simulink library "Multibody_Parts_Lib"  (R2024a)
settings: Solver=VariableStepAuto  StartTime=0.0  StopTime=10.0  RelTol=1e-3
undefined symbols (not defined in the file or in its folder): b_gear_pd_asy, b_radius_asy, b_visc_frict_asy, bevel_angle_asy, bevel_angle_bf_asy, bevel_angle_fg_asy, f_gear_pd_asy, f_radius_asy, f_visc_frict_asy, g_radius_asy, g_visc_frict_asy, gear_ra_asy, gear_visc_frict_asy, Hand, Left, Local, pinion_pd_asy, screw_lead, worm_lead_angle_asy, worm_rad_asy, worm_visc_frict_asy, X, Y, Z
libraries: sm_lib x143, $bdroot x22, nesl_utility x16
(part 4 of 6)

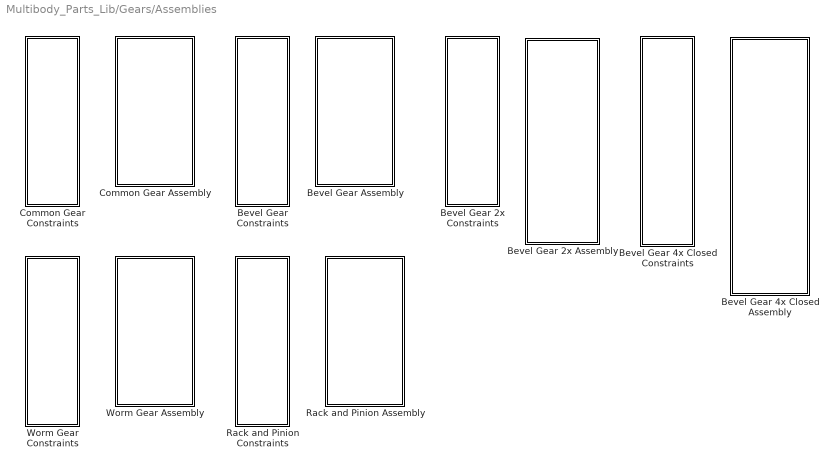
== system Multibody_Parts_Lib/Gears/Assemblies ==
  Bevel Gear Constraints : Subsystem  mask(Bevel Gear Assembly Constraints){bevel_angle=bevel_angle_asy, b_radius=b_radius_asy, f_radius=f_radius_asy, b_visc_frict=b_visc_frict_asy, f_visc_frict=f_visc_frict_asy}
      mask prompts: bevel_angle "Angle Between Shafts (deg)"
      mask help: Model connects all required constraints for a bevel gear assembly. Contains two Revolute Joints and a Bevel Gear Constraint, all positioned and oriented according to the Bevel Gear Constraint requirements.
      mask DialogControl Control3 Prompt: Gear B
      mask DialogControl Control4 Prompt: Gear F
      mask DialogControl Control5 Prompt: Gear Radius (m)
      mask DialogControl Control6 Prompt: Bearing Friction N*m/(deg/s)
  Bevel Gear 2x Assembly : Subsystem  Tag=PublishSubsystem  mask(Double Bevel Gear Assembly){bevel_angle_bf_asy=35, bevel_angle_fg_asy=35, b_cone_angle_asy=35/2, b_radius_asy=0.125, f_radius_asy=0.095, g_radius_asy=0.125, b_thickness_asy=0.02, f_thickness_asy=0.02, g_thickness_asy=0.02, b_hole_radius_asy=0.02, f_hole_radius_asy=0.02, g_hole_radius_asy=0.02, b_rho_asy=7000, f_rho_asy=7000, g_rho_asy=7000, b_clr_asy=[0.0 0.4 0.6], f_clr_asy=[0.6 0.6 0.6], g_clr_asy=[0.4 0.8 0.8], b_opc_asy=1, f_opc_asy=1, g_opc_asy=1, b_visc_frict_asy=0.01, f_visc_frict_asy=0.01, g_visc_frict_asy=0.01, b_popup_markings=Two, f_popup_markings=Two, g_popup_markings=Two, b_mark_radius_range=[0.7 0.8], f_mark_radius_range=[0.7 0.8], g_mark_radius_range=[0.7 0.8], b_mark_angle_range=60, f_mark_angle_range=60, g_mark_angle_range=60, b_mark_clr=[1 1 1], f_mark_clr=[1 1 1], g_mark_clr=[1 1 1]}
      mask prompts: bevel_angle_bf_asy "Angle Between Shafts B, F (deg)"; bevel_angle_fg_asy "Angle Between Shafts F, G (deg)"; b_cone_angle_asy "Cone Angle, Gear B (deg)"
      mask help: Models a gear assembly with three gears whose shafts may be oriented at an arbitrary angles. This assembly contains three gears constrained by three Revolute joints and two Bevel Gear Constraints.
      mask init:
      | set_param([gcb '/Gear B'],'popup_markings',get_param(gcb,'b_popup_markings'));
      | set_param([gcb '/Gear F'],'popup_markings',get_param(gcb,'f_popup_markings'));
      mask TypeOptions b_popup_markings: None | One | Two
      mask Callback b_popup_markings:
      | maskObj = Simulink.Mask.get(gcb);
      | mkrr_h = maskObj.getParameter('b_mark_radius_range');
      | mkab_h = maskObj.getParameter('b_mark_angle_range');
      | mkcl_h = maskObj.getParameter('b_mark_clr');
      | if strcmp(get_param(gcb,'b_popup_markings'),'None')
      |     mkrr_h.Visible = 'off';
      |     mkab_h.Visible = 'off';
      |     mkcl_h.Visible = 'off';
      | else
      |     mkrr_h.Visible = 'on';
      |     mkab_h.Visible = 'on';
      |     mkcl_h.Visible = 'on';
      | end
      | clear maskObj mkrr_h mkab_h mkcl_h
      mask TypeOptions f_popup_markings: None | One | Two
      mask Callback f_popup_markings:
      | maskObj = Simulink.Mask.get(gcb);
      | mkrr_h = maskObj.getParameter('f_mark_radius_range');
      | mkab_h = maskObj.getParameter('f_mark_angle_range');
      | mkcl_h = maskObj.getParameter('f_mark_clr');
      | if strcmp(get_param(gcb,'f_popup_markings'),'None')
      |     mkrr_h.Visible = 'off';
      |     mkab_h.Visible = 'off';
      |     mkcl_h.Visible = 'off';
      | else
      |     mkrr_h.Visible = 'on';
      |     mkab_h.Visible = 'on';
      |     mkcl_h.Visible = 'on';
      | end
      | clear maskObj mkrr_h mkab_h mkcl_h
      mask TypeOptions g_popup_markings: None | One | Two
      mask Callback g_popup_markings:
      | maskObj = Simulink.Mask.get(gcb);
      | mkrr_h = maskObj.getParameter('g_mark_radius_range');
      | mkab_h = maskObj.getParameter('g_mark_angle_range');
      | mkcl_h = maskObj.getParameter('g_mark_clr');
      | if strcmp(get_param(gcb,'g_popup_markings'),'None')
      |     mkrr_h.Visible = 'off';
      |     mkab_h.Visible = 'off';
      |     mkcl_h.Visible = 'off';
      | else
      |     mkrr_h.Visible = 'on';
      |     mkab_h.Visible = 'on';
      |     mkcl_h.Visible = 'on';
      | end
      | clear maskObj mkrr_h mkab_h mkcl_h
      mask DialogControl Control3 Prompt: (Add text here)
      mask DialogControl Control2 Prompt: Gear B
      mask DialogControl Control4 Prompt: Gear F
      mask DialogControl Control17 Prompt: Gear G
      mask DialogControl Control5 Prompt: Gear Radius (m)
      mask DialogControl Control6 Prompt: Thickness (m)
      mask DialogControl Control7 Prompt: Hole Radius (m)
      mask DialogControl Control10 Prompt: Density (kg/m^3)
      mask DialogControl Control11 Prompt: Color [RGB]
      mask DialogControl Control18 Prompt: Opacity (0-1)
      mask DialogControl Control8 Prompt: Bearing Friction N*m/(deg/s)
      mask DialogControl Container3 Prompt: Gear Markings
      mask DialogControl Control13 Prompt: Show Marking
      mask DialogControl text_radial_range Prompt: Radial Range (0-1)
      mask DialogControl text_sweep_angle Prompt: Sweep Angle (0-180)
      mask DialogControl text_mark_clr Prompt: Color [RGB]
      mask Display: image('sm_bevel_gear_2x_assembly.png')
  Bevel Gear 2x Constraints : Subsystem  mask(Double Bevel Gear Assembly Constraints){bevel_angle_bf=bevel_angle_bf_asy, bevel_angle_fg=bevel_angle_fg_asy, b_radius=b_radius_asy, f_radius=f_radius_asy, g_radius=g_radius_asy, b_visc_frict=b_visc_frict_asy, f_visc_frict=f_visc_frict_asy, g_visc_frict=g_visc_frict_asy}
      mask prompts: bevel_angle_bf "Angle Between Shaft B, F (deg)"; bevel_angle_fg "Angle Between Shaft F, G (deg)"
      mask help: Model connects all required constraints for a double bevel gear assembly. Contains three Revolute Joints and two Bevel Gear Constraints, all positioned and oriented according to the Bevel Gear Constraint requirements.
      mask DialogControl Control3 Prompt: Gear B
      mask DialogControl Control4 Prompt: Gear F
      mask DialogControl Control7 Prompt: Gear G
      mask DialogControl Control5 Prompt: Gear Radius (m)
      mask DialogControl Control6 Prompt: Bearing Friction N*m/(deg/s)
  Bevel Gear 4x Closed Assembly : Subsystem  Tag=PublishSubsystem  mask(Bevel Gear Assembly){bevel_angle_asy=90, b_cone_angle_asy=90/2, b_radius_asy=0.125, f_radius_asy=0.175, b_thickness_asy=0.02, f_thickness_asy=0.02, b_hole_radius_asy=0.02, f_hole_radius_asy=0.02, b_rho_asy=7000, f_rho_asy=7000, b_clr_asy=[0.0 0.4 0.6], f_clr_asy=[0.6 0.6 0.6], b_opc_asy=1, f_opc_asy=1, b_visc_frict_asy=0.01, f_visc_frict_asy=0.01, b_popup_markings=Two, f_popup_markings=Two, b_mark_radius_range=[0.7 0.8], f_mark_radius_range=[0.7 0.8], b_mark_angle_range=60, f_mark_angle_range=60, b_mark_clr=[1 1 1], f_mark_clr=[1 1 1]}
      mask prompts: bevel_angle_asy "Angle Between Shafts (deg)"; b_cone_angle_asy "Cone Angle, Gear B (deg)"
      mask help: Models a gear assembly with two gears whose shafts may be oriented at an arbitrary angle. This assembly contains two gears constrained by two Revolute joints and a Bevel Gear Constraint.
      mask init:
      | set_param([gcb '/Gear B1'],'popup_markings',get_param(gcb,'b_popup_markings'));
      | set_param([gcb '/Gear F1'],'popup_markings',get_param(gcb,'f_popup_markings'));
      | set_param([gcb '/Gear B2'],'popup_markings',get_param(gcb,'b_popup_markings'));
      | set_param([gcb '/Gear F2'],'popup_markings',get_param(gcb,'f_popup_markings'));
      mask TypeOptions b_popup_markings: None | One | Two
      mask Callback b_popup_markings:
      | maskObj = Simulink.Mask.get(gcb);
      | mkrr_h = maskObj.getParameter('b_mark_radius_range');
      | mkab_h = maskObj.getParameter('b_mark_angle_range');
      | mkcl_h = maskObj.getParameter('b_mark_clr');
      | if strcmp(get_param(gcb,'b_popup_markings'),'None')
      |     mkrr_h.Visible = 'off';
      |     mkab_h.Visible = 'off';
      |     mkcl_h.Visible = 'off';
      | else
      |     mkrr_h.Visible = 'on';
      |     mkab_h.Visible = 'on';
      |     mkcl_h.Visible = 'on';
      | end
      | clear maskObj mkrr_h mkab_h mkcl_h
      mask TypeOptions f_popup_markings: None | One | Two
      mask Callback f_popup_markings:
      | maskObj = Simulink.Mask.get(gcb);
      | mkrr_h = maskObj.getParameter('f_mark_radius_range');
      | mkab_h = maskObj.getParameter('f_mark_angle_range');
      | mkcl_h = maskObj.getParameter('f_mark_clr');
      | if strcmp(get_param(gcb,'f_popup_markings'),'None')
      |     mkrr_h.Visible = 'off';
      |     mkab_h.Visible = 'off';
      |     mkcl_h.Visible = 'off';
      | else
      |     mkrr_h.Visible = 'on';
      |     mkab_h.Visible = 'on';
      |     mkcl_h.Visible = 'on';
      | end
      | clear maskObj mkrr_h mkab_h mkcl_h
      mask DialogControl Control3 Prompt: (Add text here)
      mask DialogControl Control2 Prompt: Gear B
      mask DialogControl Control4 Prompt: Gear F
      mask DialogControl Control5 Prompt: Gear Radius (m)
      mask DialogControl Control6 Prompt: Thickness (m)
      mask DialogControl Control7 Prompt: Hole Radius (m)
      mask DialogControl Control10 Prompt: Density (kg/m^3)
      mask DialogControl Control11 Prompt: Color [RGB]
      mask DialogControl Control17 Prompt: Opacity (0-1)
      mask DialogControl Control8 Prompt: Bearing Friction N*m/(deg/s)
      mask DialogControl Container3 Prompt: Gear Markings
      mask DialogControl Control13 Prompt: Show Marking
      mask DialogControl text_radial_range Prompt: Radial Range (0-1)
      mask DialogControl text_sweep_angle Prompt: Sweep Angle (0-180)
      mask DialogControl text_mark_clr Prompt: Color [RGB]
      mask Display: image('sm_bevel_gear_4x_closed_assembly.png')
  Bevel Gear 4x Closed Constraints : Subsystem  mask(Bevel Gear Assembly Constraints){bevel_angle=bevel_angle_asy, b_radius=b_radius_asy, f_radius=f_radius_asy, b_visc_frict=b_visc_frict_asy, f_visc_frict=f_visc_frict_asy}
      mask prompts: bevel_angle "Angle Between Shafts (deg)"
      mask help: Model connects all required constraints for a bevel gear assembly. Contains two Revolute Joints and a Bevel Gear Constraint, all positioned and oriented according to the Bevel Gear Constraint requirements.
      mask DialogControl Control3 Prompt: Gear B
      mask DialogControl Control4 Prompt: Gear F
      mask DialogControl Control5 Prompt: Gear Radius (m)
      mask DialogControl Control6 Prompt: Bearing Friction N*m/(deg/s)
  Bevel Gear Assembly : Subsystem  Tag=PublishSubsystem  mask(Bevel Gear Assembly){bevel_angle_asy=45, b_cone_angle_asy=45/2, b_radius_asy=0.125, f_radius_asy=0.175, b_thickness_asy=0.02, f_thickness_asy=0.02, b_hole_radius_asy=0.02, f_hole_radius_asy=0.02, b_rho_asy=7000, f_rho_asy=7000, b_clr_asy=[0.0 0.4 0.6], f_clr_asy=[0.6 0.6 0.6], b_opc_asy=1, f_opc_asy=1, b_visc_frict_asy=0.01, f_visc_frict_asy=0.01, b_popup_markings=Two, f_popup_markings=Two, b_mark_radius_range=[0.7 0.8], f_mark_radius_range=[0.7 0.8], b_mark_angle_range=60, f_mark_angle_range=60, b_mark_clr=[1 1 1], f_mark_clr=[1 1 1]}
      mask prompts: bevel_angle_asy "Angle Between Shafts (deg)"; b_cone_angle_asy "Cone Angle, Gear B (deg)"
      mask help: Models a gear assembly with two gears whose shafts may be oriented at an arbitrary angle. This assembly contains two gears constrained by two Revolute joints and a Bevel Gear Constraint.
      mask init:
      | set_param([gcb '/Gear B'],'popup_markings',get_param(gcb,'b_popup_markings'));
      | set_param([gcb '/Gear F'],'popup_markings',get_param(gcb,'f_popup_markings'));
      mask TypeOptions b_popup_markings: None | One | Two
      mask Callback b_popup_markings:
      | maskObj = Simulink.Mask.get(gcb);
      | mkrr_h = maskObj.getParameter('b_mark_radius_range');
      | mkab_h = maskObj.getParameter('b_mark_angle_range');
      | mkcl_h = maskObj.getParameter('b_mark_clr');
      | if strcmp(get_param(gcb,'b_popup_markings'),'None')
      |     mkrr_h.Visible = 'off';
      |     mkab_h.Visible = 'off';
      |     mkcl_h.Visible = 'off';
      | else
      |     mkrr_h.Visible = 'on';
      |     mkab_h.Visible = 'on';
      |     mkcl_h.Visible = 'on';
      | end
      | clear maskObj mkrr_h mkab_h mkcl_h
      mask TypeOptions f_popup_markings: None | One | Two
      mask Callback f_popup_markings:
      | maskObj = Simulink.Mask.get(gcb);
      | mkrr_h = maskObj.getParameter('f_mark_radius_range');
      | mkab_h = maskObj.getParameter('f_mark_angle_range');
      | mkcl_h = maskObj.getParameter('f_mark_clr');
      | if strcmp(get_param(gcb,'f_popup_markings'),'None')
      |     mkrr_h.Visible = 'off';
      |     mkab_h.Visible = 'off';
      |     mkcl_h.Visible = 'off';
      | else
      |     mkrr_h.Visible = 'on';
      |     mkab_h.Visible = 'on';
      |     mkcl_h.Visible = 'on';
      | end
      | clear maskObj mkrr_h mkab_h mkcl_h
      mask DialogControl Control3 Prompt: (Add text here)
      mask DialogControl Control2 Prompt: Gear B
      mask DialogControl Control4 Prompt: Gear F
      mask DialogControl Control5 Prompt: Gear Radius (m)
      mask DialogControl Control6 Prompt: Thickness (m)
      mask DialogControl Control7 Prompt: Hole Radius (m)
      mask DialogControl Control10 Prompt: Density (kg/m^3)
      mask DialogControl Control11 Prompt: Color [RGB]
      mask DialogControl Control17 Prompt: Opacity (0-1)
      mask DialogControl Control8 Prompt: Bearing Friction N*m/(deg/s)
      mask DialogControl Container3 Prompt: Gear Markings
      mask DialogControl Control13 Prompt: Show Marking
      mask DialogControl text_radial_range Prompt: Radial Range (0-1)
      mask DialogControl text_sweep_angle Prompt: Sweep Angle (0-180)
      mask DialogControl text_mark_clr Prompt: Color [RGB]
      mask Display: image('sm_bevel_gear_assembly.png')
  Common Gear Constraints : Subsystem  mask(Common Gear Assembly Constraints){popup_gear_type=External, b_gear_pd=b_gear_pd_asy, f_gear_pd=f_gear_pd_asy, b_visc_frict=b_visc_frict_asy, f_visc_frict=f_visc_frict_asy}
      mask prompts: popup_gear_type "Gear Type"
      mask help: Model connects all required constraints for a common gear assembly. Contains two Revolute Joints and a Common Gear Constraint, all oriented and positioned according to the Common Gear Constraint requirements.
      mask init:
      | gear_constr_type = get_param(gcb,'popup_gear_type');
      | set_param([gcb '/Common Gear Constraint'],'GearType',gear_constr_type);
      | if(strcmpi(gear_constr_type,'External'))
      |     gear_axis_offset = (f_gear_pd+b_gear_pd)/2;
      | else
      |     gear_axis_offset = (f_gear_pd-b_gear_pd)/2;
      | end
      mask TypeOptions popup_gear_type: External | Internal
      mask DialogControl Control3 Prompt: Gear B
      mask DialogControl Control4 Prompt: Gear F
      mask DialogControl Control5 Prompt: Pitch Diameter (m)
      mask DialogControl Control6 Prompt: Bearing Friction N*m/(deg/s)
  Common Gear Assembly : Subsystem  Tag=PublishSubsystem  mask(Common Gear Assembly){b_gear_pd_asy=0.125, f_gear_pd_asy=0.25, b_gear_nt=12, f_gear_nt=24, b_gear_th=0.02, f_gear_th=0.02, f_popup_gear_type=External, b_gear_rh=0.01, f_gear_rht=0.01, b_gear_offset_angle=0, f_gear_offset_angle=360/24/2, b_gear_rho=7000, f_gear_rho=7000, b_gear_clr=[0.0 0.4 0.6], f_gear_clr=[0.6 0.6 0.6], b_gear_opc=1, f_gear_opc=1, popup_ad_dd_asy=Specify, b_gear_ad=0.125/12, f_gear_ad=0.25/24, b_gear_dd=1.157*0.125/12, f_gear_dd=1.157*0.25/24, b_visc_frict_asy=0.01, f_visc_frict_asy=0.01, b_popup_markings=Two, f_popup_markings=Two, b_mark_radius_range=[0.6 0.7], f_mark_radius_range=[0.7 0.8], b_mark_angle_range=60, f_mark_angle_range=60, b_mark_color=[1 1 1], f_mark_color=[1 1 1]}
      mask prompts: popup_ad_dd_asy "Addendum, Dedendum"
      mask help: Models a gear assembly with two gears whose shafts are parallel. This assembly contains two gears constrained by two revolute joints and a common gear constraint. It can be configured to model an external gear or an internal gear pair.
      mask init:
      | set_param([gcb '/Gear B'],'popup_markings',get_param(gcb,'b_popup_markings'));
      | set_param([gcb '/Gear F'],'popup_markings',get_param(gcb,'f_popup_markings'));
      | 
      | gear_constr_type = get_param(gcb,'f_popup_gear_type');
      | 
      | set_param([gcb '/Gear F'],...
      |     'popup_gear_type',gear_constr_type,...
      |     'popup_ad_dd',get_param(gcb,'popup_ad_dd_asy'));
      | 
      | set_param([gcb '/Gear B'],...
      |     'popup_ad_dd',get_param(gcb,'popup_ad_dd_asy'));
      | 
      | set_param([gcb '/Constraints'],'popup_gear_type',gear_constr_type);
      mask TypeOptions f_popup_gear_type: External | Internal
      mask Callback f_popup_gear_type:
      | maskObj = Simulink.Mask.get(gcb);
      | fradt_h = maskObj.getDialogControl('f_rad_text');
      | if strcmp(get_param(gcb,'f_popup_gear_type'),'External')
      |     fradt_h.Prompt = 'Hole Radius (m)';
      | else
      |     fradt_h.Prompt = 'External Radius (m)';
      | end
      | clear maskObj fradt_h
      mask TypeOptions popup_ad_dd_asy: Default | Specify
      mask Callback popup_ad_dd_asy:
      | maskObj = Simulink.Mask.get(gcb);
      | addd_h = maskObj.getDialogControl('container_ad_dd');
      | if strcmp(get_param(gcb,'popup_ad_dd_asy'),'Default')
      |     addd_h.Visible = 'off';
      | else
      |     addd_h.Visible = 'on';
      | end
      | clear maskObj addd_h
      mask TypeOptions b_popup_markings: None | One | Two
      mask Callback b_popup_markings:
      | maskObj = Simulink.Mask.get(gcb);
      | mkrr_h = maskObj.getParameter('b_mark_radius_range');
      | mkab_h = maskObj.getParameter('b_mark_angle_range');
      | mkcl_h = maskObj.getParameter('b_mark_color');
      | if strcmp(get_param(gcb,'b_popup_markings'),'None')
      |     mkrr_h.Visible = 'off';
      |     mkab_h.Visible = 'off';
      |     mkcl_h.Visible = 'off';
      | else
      |     mkrr_h.Visible = 'on';
      |     mkab_h.Visible = 'on';
      |     mkcl_h.Visible = 'on';
      | end
      | clear maskObj mkrr_h mkab_h mkcl_h
      mask TypeOptions f_popup_markings: None | One | Two
      mask Callback f_popup_markings:
      | maskObj = Simulink.Mask.get(gcb);
      | mkrr_h = maskObj.getParameter('f_mark_radius_range');
      | mkab_h = maskObj.getParameter('f_mark_angle_range');
      | mkcl_h = maskObj.getParameter('f_mark_color');
      | if strcmp(get_param(gcb,'f_popup_markings'),'None')
      |     mkrr_h.Visible = 'off';
      |     mkab_h.Visible = 'off';
      |     mkcl_h.Visible = 'off';
      | else
      |     mkrr_h.Visible = 'on';
      |     mkab_h.Visible = 'on';
      |     mkcl_h.Visible = 'on';
      | end
      | clear maskObj mkrr_h mkab_h mkcl_h
      mask DialogControl Control3 Prompt: (Add text here)
      mask DialogControl Control2 Prompt: Gear B
      mask DialogControl Control4 Prompt: Gear F
      mask DialogControl Control5 Prompt: Pitch Diameter (m)
      mask DialogControl Control17 Prompt: Number of Teeth
      mask DialogControl Control6 Prompt: Thickness (m)
      mask DialogControl Control18 Prompt: Gear Type
      mask DialogControl Control19 Prompt: External
      mask DialogControl Control26 Prompt: (Add text here)
      mask DialogControl b_rad_text Prompt: Hole Radius (m)
      mask DialogControl f_rad_text Prompt: Hole Radius (m)
      mask DialogControl Control28 Prompt: (Add text here)
      mask DialogControl Control31 Prompt: Offset Angle (deg)
      mask DialogControl Control10 Prompt: Density (kg/m^3)
      mask DialogControl Control11 Prompt: Color [RGB]
      mask DialogControl Control33 Prompt: Opacity (0-1)
      mask DialogControl Control23 Prompt: Addendum (m)
      mask DialogControl Control24 Prompt: Dedendum (m)
      mask DialogControl Control8 Prompt: Bearing Friction N*m/(deg/s)
      mask DialogControl Container3 Prompt: Gear Markings
      mask DialogControl Control13 Prompt: Show Marking
      mask DialogControl text_radial_range Prompt: Radial Range (0-1)
      mask DialogControl text_sweep_angle Prompt: Sweep Angle (0-180)
      mask DialogControl text_mark_clr Prompt: Color [RGB]
      mask Display:
      | if(strcmpi(gear_constr_type,'External'))
      |     image('sm_common_gear_assembly_external.png');
      | else
      |     image('sm_common_gear_assembly_internal.png');
      | end
  Rack and Pinion Constraints : Subsystem  mask(Rack and Pinion Assembly Constraints){pinion_pd=pinion_pd_asy, pinion_visc_frict=0, rack_visc_frict=0}
      mask prompts: pinion_pd "Pitch Diameter (m)"; pinion_visc_frict "Pinion Bearing Friction N*m/(deg/s)"; rack_visc_frict "Rack Bearing Friction (N/(m/s))"
      mask help: Model connects all required constraints for a rack and pinion assembly. Contains one Prismatic Joint, one Revolute Joint, and a Rack and Pinion Constraint, all oriented and positioned according to the Rack and Pinion Constraint requirements.
  Rack and Pinion Assembly : Subsystem  mask(Rack and Pinion Assembly){pinion_pd_asy=0.5, pinion_nt_asy=30, pinion_th_asy=0.02, pinion_rh_asy=0.02, pinion_rho_asy=7000, pinion_clr_asy=[0 0.4 0.7], pinion_opc_asy=1, p_popup_ad_dd=Default, pinion_ad_asy=0.5/30, pinion_dd_asy=1.157*0.5/30, pinion_visc_frict_asy=0, p_popup_markings=Two, p_mark_radius_range=[0.7 0.8], p_mark_angle_range=120, p_mark_color=[1 1 1], rack_tp_asy=0.052, rack_nt_asy=29, rack_tb_asy=0.02, rack_th_asy=0.02, rack_rho_asy=7000, rack_clr_asy=[0.5 0.5 0.5], rack_opc_asy=1, r_popup_ad_dd=Default, rack_ad_asy=0.052/29, rack_dd_asy=1.157*0.052/29, rack_visc_frict_asy=0}
      mask prompts: pinion_pd_asy "Pitch Diameter (m)"; pinion_nt_asy "Number of Teeth"; pinion_th_asy "Gear Thickness (m)"; pinion_rh_asy "Hole Radius (m)"; pinion_rho_asy "Density (kg/m^3)"; pinion_clr_asy "Color [RGB]"; pinion_opc_asy "Opacity (0-1):"; p_popup_ad_dd "Addendum, Dedendum"; pinion_ad_asy "Addendum (m)"; pinion_dd_asy "Dedendum (m)"; pinion_visc_frict_asy "Pinion Bearing Friction N*m/(deg/s)"; p_popup_markings "Show Markings"; p_mark_radius_range "Radial Range [min max] (0-1)"; p_mark_angle_range "Sweep Angle [0-180] (deg)"; p_mark_color "Color [RGB]"; rack_tp_asy "Teeth Pitch (m)"; rack_nt_asy "Number of Teeth"; rack_tb_asy "Thickness of Rack Base (m)"; rack_th_asy "Thickness of Rack (m)"; rack_rho_asy "Density (kg/m^3)"; rack_clr_asy "Color [RGB]"; rack_opc_asy "Opacity (0-1):"; r_popup_ad_dd "Addendum, Dedendum"; rack_ad_asy "Addendum (m)"; rack_dd_asy "Dedendum (m)"; rack_visc_frict_asy "Rack Bearing Friction (N/(m/s))"
      mask help: Models a gear assembly with a spur gear and a toothed bar. This assembly contains a gear and a rack constrained by one Revolute Joint, one Prismatic Joint, and a Rack and Pinion Constraint.
      mask init:
      | set_param([gcb '/Pinion'],...
      |     'popup_gear_type','External',...
      |     'popup_ad_dd',get_param(gcb,'p_popup_ad_dd'),...
      |     'popup_markings',get_param(gcb,'p_popup_markings'));
      | 
      | set_param([gcb '/Rack'],...
      |     'popup_ad_dd',get_param(gcb,'r_popup_ad_dd'));
      mask TypeOptions p_popup_ad_dd: Default | Specify
      mask Callback p_popup_ad_dd:
      | maskObj = Simulink.Mask.get(gcb);
      | gad_h = maskObj.getParameter('pinion_ad_asy');
      | gdd_h = maskObj.getParameter('pinion_dd_asy');
      | if strcmp(get_param(gcb,'p_popup_ad_dd'),'Default')
      |     gad_h.Visible = 'off';
      |     gdd_h.Visible = 'off';
      | else
      |     gad_h.Visible = 'on';
      |     gdd_h.Visible = 'on';
      | end
      | clear maskObj gad_h gdd_h
      mask TypeOptions p_popup_markings: None | One | Two
      mask Callback p_popup_markings:
      | maskObj = Simulink.Mask.get(gcb);
      | mkc_h = maskObj.getDialogControl('container_markings');
      | if strcmp(get_param(gcb,'p_popup_markings'),'None')
      |     mkc_h.Visible = 'off';
      | else
      |     mkc_h.Visible = 'on';
      | end
      | clear maskObj mkc_h
      mask TypeOptions r_popup_ad_dd: Default | Specify
      mask Callback r_popup_ad_dd:
      | maskObj = Simulink.Mask.get(gcb);
      | rad_h = maskObj.getParameter('rack_ad_asy');
      | rdd_h = maskObj.getParameter('rack_dd_asy');
      | if strcmp(get_param(gcb,'r_popup_ad_dd'),'Default')
      |     rad_h.Visible = 'off';
      |     rdd_h.Visible = 'off';
      | else
      |     rad_h.Visible = 'on';
      |     rdd_h.Visible = 'on';
      | end
      | clear maskObj rad_h rdd_h
      mask DialogControl pinion_tab Prompt: Pinion
      mask DialogControl rack_tab Prompt: Rack
      mask Display: image('sm_rack_and_pinion_assembly.png')
  Worm Gear Constraints : Subsystem  mask(Worm Gear Assembly Constraints){popup_worm_dir=Left-Hand, worm_lead_angle=worm_lead_angle_asy, worm_rad=worm_rad_asy, gear_rad=gear_ra_asy, worm_visc_frict=worm_visc_frict_asy, gear_visc_frict=gear_visc_frict_asy}
      mask prompts: popup_worm_dir "Worm Direction"; worm_lead_angle "Worm Lead Angle (deg)"; worm_rad "Worm Radius (m)"; gear_rad "Gear Radius (m)"; worm_visc_frict "Worm Bearing Friction (N*m/(deg/s))"; gear_visc_frict "Gear Bearing Friction (N*m/(deg/s))"
      mask help: Model connects all required constraints for a worm gear assembly. Contains two Revolute Joints and a Worm Gear Constraint, all positioned and oriented according to the Worm Gear Constraint requirements.
      mask init:
      | if(strcmpi(get_param(gcb,'popup_worm_dir'),'Right-Hand'))
      | set_param([gcb '/Worm and Gear Constraint'],...
      |     'WormDirection','RightHand')
      | else
      |     set_param([gcb '/Worm and Gear Constraint'],...
      |     'WormDirection','LeftHand')
      | end
      mask TypeOptions popup_worm_dir: Right-Hand | Left-Hand
  Worm Gear Assembly : Subsystem  mask(Worm Gear Assembly){popup_worm_dir_asy=Left-Hand, worm_lead_angle_asy=4.2, gear_ra_asy=37.5e-3, gear_th_asy=9e-3, gear_hr_asy=5e-3, gear_rho_asy=7000, gear_clr_asy=[0.6 0.6 0.6], gear_opc_asy=1, gear_visc_frict_asy=1e-2, g_popup_markings=Two, g_mark_radius_range=[0.7 0.9], g_mark_angle_range=60, g_mark_color=[1 1 1], worm_rad_asy=8.5e-3, worm_len_asy=85e-3, worm_rho_asy=7000, worm_color_asy=[0.0 0.4 0.6], worm_opc_asy=1, worm_visc_frict_asy=1e-2, w_popup_markings=Two, w_mark_radius_range=[0.5 1.01], w_mark_length_range=1.005, w_mark_angle_range=30, w_mark_color=[1 1 1]}
      mask prompts: popup_worm_dir_asy "Worm Direction"; worm_lead_angle_asy "Worm Lead Angle (deg)"; gear_ra_asy "Radius (m):"; gear_th_asy "Thickness (m):"; gear_hr_asy "Hole Radius (m):"; gear_rho_asy "Density (kg/m^3):"; gear_clr_asy "Color [RGB]:"; gear_opc_asy "Opacity (0-1):"; gear_visc_frict_asy "Bearing Friction N*m/(deg/s)"; g_popup_markings "Show Markings"; g_mark_radius_range "Radial Range [min max] (0-1)"; g_mark_angle_range "Sweep Angle [0-180] (deg)"; g_mark_color "Color [RGB]"; worm_rad_asy "Radius (m)"; worm_len_asy "Length (m)"; worm_rho_asy "Density (kg/m^3)"; worm_color_asy "Color [RGB]"; worm_opc_asy "Opacity (0-1):"; worm_visc_frict_asy "Bearing Friction N*m/(deg/s)"; w_popup_markings "Show Markings"; w_mark_radius_range "Radial Range [min max] (0-1.1)"; w_mark_length_range "Length Range (0-1.1)"; w_mark_angle_range "Sweep Angle [0-180] (deg)"; w_mark_color "Color [RGB]"
      mask help: Models a gear assembly with two gears whose axes are perpendicular but do not intersect. This assembly contains two gears constrained by two Revolute Joints and a Worm Gear Constraint.
      mask init:
      | set_param([gcb '/Gear'],'popup_markings',get_param(gcb,'g_popup_markings'));
      | set_param([gcb '/WormB'],'popup_markings',get_param(gcb,'w_popup_markings'));
      | set_param([gcb '/WormF'],'popup_markings',get_param(gcb,'w_popup_markings'));
      | set_param([gcb '/Constraints'],'popup_worm_dir',get_param(gcb,'popup_worm_dir_asy'));
      mask TypeOptions popup_worm_dir_asy: Right-Hand | Left-Hand
      mask TypeOptions g_popup_markings: None | One | Two
      mask Callback g_popup_markings:
      | maskObj = Simulink.Mask.get(gcb);
      | mkc_h = maskObj.getDialogControl('g_container_markings');
      | if strcmp(get_param(gcb,'g_popup_markings'),'None')
      |     mkc_h.Visible = 'off';
      | else
      |     mkc_h.Visible = 'on';
      | end
      | clear maskObj mkc_h
      mask TypeOptions w_popup_markings: None | One | Two
      mask Callback w_popup_markings:
      | maskObj = Simulink.Mask.get(gcb);
      | mkc_h = maskObj.getDialogControl('w_container_markings');
      | if strcmp(get_param(gcb,'w_popup_markings'),'None')
      |     mkc_h.Visible = 'off';
      | else
      |     mkc_h.Visible = 'on';
      | end
      | clear maskObj mkc_h
      mask DialogControl Gear Prompt: Gear
      mask DialogControl Worm Prompt: Worm
      mask Display: image('sm_worm_gear_assembly.png')

== system Multibody_Parts_Lib/Gears/Bevel Gear ==
  Gear : sm_lib/Body Elements/Revolved Solid  RevolutionCrossSection=gear_xsec  RevolutionCrossSectionUnits=m  RevolutionExtent=Full  RevolutionAngle=355  RevolutionAngleUnits=deg  ExportConvexHullGeometry=off  InertiaType=CalculateFromGeometry  BasedOnType=Density  Density=gear_rho  DensityUnits=kg/(m^3)  Mass=1  MassUnits=kg  CenterOfMass=[0 0 0]  CenterOfMassUnits=m  MomentsOfInertia=[1 1 1]  MomentsOfInertiaUnits=kg*m^2  ProductsOfInertia=[0 0 0]  ProductsOfInertiaUnits=kg*m^2  GraphicType=FromGeometry  MarkerShape=Sphere  MarkerSize=10  GraphicVisPropType=SimpleVisualProperties  GraphicDiffuseColor=gear_clr  GraphicOpacity=gear_opc  GraphicSpecularColor=[0.5 0.5 0.5 1.0]  GraphicAmbientColor=[0.15 0.15 0.15 1.0]  GraphicEmissiveColor=[0.0 0.0 0.0 1.0]  GraphicShininess=75  DoExposeReferenceFrame=on  SerializedFrames=<Frames/>
  Mark1 : sm_lib/Body Elements/Revolved Solid  RevolutionCrossSection=mark_xsec  RevolutionCrossSectionUnits=m  RevolutionExtent=Custom  RevolutionAngle=mark_angle_range  RevolutionAngleUnits=deg  ExportConvexHullGeometry=off  InertiaType=CalculateFromGeometry  BasedOnType=Density  Density=0  DensityUnits=kg/m^3  Mass=1  MassUnits=kg  CenterOfMass=[0 0 0]  CenterOfMassUnits=m  MomentsOfInertia=[1 1 1]  MomentsOfInertiaUnits=kg*m^2  ProductsOfInertia=[1 1 1]  ProductsOfInertiaUnits=kg*m^2  GraphicType=FromGeometry  MarkerShape=Sphere  MarkerSize=10  GraphicVisPropType=SimpleVisualProperties  GraphicDiffuseColor=mark_color  GraphicOpacity=mark_1_opc  GraphicSpecularColor=[0.5 0.5 0.5 1.0]  GraphicAmbientColor=[0.15 0.15 0.15 1.0]  GraphicEmissiveColor=[0.0 0.0 0.0 1.0]  GraphicShininess=75  DoExposeReferenceFrame=on  SerializedFrames=<Frames/>
  Mark2 : sm_lib/Body Elements/Revolved Solid  RevolutionCrossSection=mark_xsec  RevolutionCrossSectionUnits=m  RevolutionExtent=Custom  RevolutionAngle=mark_angle_range  RevolutionAngleUnits=deg  ExportConvexHullGeometry=off  InertiaType=CalculateFromGeometry  BasedOnType=Density  Density=0  DensityUnits=kg/m^3  Mass=1  MassUnits=kg  CenterOfMass=[0 0 0]  CenterOfMassUnits=m  MomentsOfInertia=[1 1 1]  MomentsOfInertiaUnits=kg*m^2  ProductsOfInertia=[1 1 1]  ProductsOfInertiaUnits=kg*m^2  GraphicType=FromGeometry  MarkerShape=Sphere  MarkerSize=10  GraphicVisPropType=SimpleVisualProperties  GraphicDiffuseColor=mark_color  GraphicOpacity=mark_2_opc  GraphicSpecularColor=[0.5 0.5 0.5 1.0]  GraphicAmbientColor=[0.15 0.15 0.15 1.0]  GraphicEmissiveColor=[0.0 0.0 0.0 1.0]  GraphicShininess=75  DoExposeReferenceFrame=on  SerializedFrames=<Frames/>
  Transform Mark 2 : sm_lib/Frames and Transforms/Rigid Transform  RotationMethod=StandardAxis  FollAlignAxisA=+X  BaseAlignAxisA=+Y  FollAlignAxisB=+Y  BaseAlignAxisB=+Z  RotationStandardAxis=+Z  RotationAngle=180  RotationAngleUnits=deg  RotationArbitraryAxis=[0 0 1]  RotationSequenceAxes=FollowerAxes  RotationSequence=XYX  RotationSequenceAngles=[0 0 0]  RotationSequenceAnglesUnits=deg  RotationMatrix=[1 0 0; 0 1 0; 0 0 1]  Quaternion=[1 0 0 0]  TranslationMethod=None  TranslationCartesianOffset=[0 0 0]  TranslationCartesianOffsetUnits=m  TranslationStandardAxis=+Z  TranslationStandardOffset=0  TranslationStandardOffsetUnits=m  TranslationROffset=0  TranslationROffsetUnits=m  TranslationThetaOffset=0  TranslationThetaOffsetUnits=deg  TranslationZOffset=0  TranslationZOffsetUnits=m
  C : PMIOPort  Side=Right
  connections:
  Transform Mark 2/RConn1 -- Mark2/RConn1
  Mark1/RConn1 -- Gear/RConn1 -- C/RConn1 -- Transform Mark 2/LConn1

== system Multibody_Parts_Lib/Gears/Forces ==
  Lead Screw Friction : Subsystem  Tag=PublishSubsystem  mask(Lead Screw Friction){mu_kinetic=0.195, mu_static=0.195, vel_th=1e-3, lead=screw_lead, screw_radius=0.02, filt_const=1e-3}
      mask prompts: mu_kinetic "Coefficient of Kinetic Friction"; mu_static "Coefficient of Static Friction"; vel_th "Velocity Threshold (m/s)"; lead "Lead (m/rev)"; screw_radius "Screw Radius (m)"; filt_const "Low Pass Filter Constant (s)"
      mask help:
      | Models friction within a lead screw.  The constraint force within the Lead Screw Joint is used to determine the friction torque that resists the rotation of the screw.  If the coefficient of friction is higher than the tangent of the lead angle, the lead screw is non-backdriveable.
      |
      | Connect the Constraint Force Output of the Lead Screw Joint to Fc, and the rotational velocity output to the w input.
      |
      | Smaller values for Velocity Threshold and Low Pass Filter Constant makes the model closer to reality but result in a numerically stiffer system.
      mask init:
      | lead_angle = atan(lead/(2*pi*screw_radius))*180/pi;
      | set_param(gcb,'AttributesFormatString',...
      |     sprintf('%s%0.3f%s\n%s%0.3f',...
      |     'Lead Angle = ',...
      |     lead_angle,...
      |     ' deg',...
      |     'Kinetic Friction = ',...
      |     mu_kinetic));
      settings: AttributesFormatString=|
      | Lead Angle =  deg
      | Kinetic Friction = 0.195
  Lead Screw Joint : sm_lib/Joints/Lead Screw Joint  JointMode=Normal  CompositeWrenchDir=FollowerOnBase  CompositeWrenchFrame=BaseFrame  SenseConstraintForce=on  SenseConstraintTorque=off  SenseTotalForce=off  SenseTotalTorque=off  Direction=RightHand  Lead=screw_lead  LeadUnits=m/rev  PositionTargetSpecify=off  PositionTargetPriority=High  PositionTargetRotationBased=off  PositionTargetRotationValue=0  PositionTargetRotationValueUnits=deg  PositionTargetTranslationValue=0  PositionTargetTranslationValueUnits=m  VelocityTargetSpecify=off  VelocityTargetPriority=High  VelocityTargetRotationBased=off  VelocityTargetRotationValue=0  VelocityTargetRotationValueUnits=deg/s  VelocityTargetTranslationValue=0  VelocityTargetTranslationValueUnits=m/s  SenseRotationPosition=off  SenseRotationVelocity=on  SenseRotationAcceleration=off  SenseTranslationPosition=off  SenseTranslationVelocity=off  SenseTranslationAcceleration=off
      settings: AttributesFormatString=%<Direction>
  connections:
  Lead Screw Friction/LConn2 -- Lead Screw Joint/RConn2
  Lead Screw Friction/LConn1 -- Lead Screw Joint/RConn3
  Lead Screw Friction/RConn1 -- Lead Screw Joint/LConn1

== system Multibody_Parts_Lib/Gears/Gear ==
  Gear : sm_lib/Body Elements/Extruded Solid  ExtrusionType=General  PolygonNumSides=3  PolygonOuterRadius=1  PolygonOuterRadiusUnits=m  ExportEntireGeometry=off  ExtrusionCrossSection=gear_xsec  ExtrusionCrossSectionUnits=m  ExportConvexHullGeometry=off  ExtrusionLength=gear_th  ExtrusionLengthUnits=m  InertiaType=CalculateFromGeometry  BasedOnType=Density  Density=gear_rho  DensityUnits=kg/(m^3)  Mass=1  MassUnits=kg  CenterOfMass=[0 0 0]  CenterOfMassUnits=m  MomentsOfInertia=[1 1 1]  MomentsOfInertiaUnits=kg*m^2  ProductsOfInertia=[0 0 0]  ProductsOfInertiaUnits=kg*m^2  GraphicType=FromGeometry  MarkerShape=Sphere  MarkerSize=10  GraphicVisPropType=SimpleVisualProperties  GraphicDiffuseColor=gear_clr  GraphicOpacity=gear_opc  GraphicSpecularColor=[0.5 0.5 0.5 1.0]  GraphicAmbientColor=[0.15 0.15 0.15 1.0]  GraphicEmissiveColor=[0.0 0.0 0.0 1.0]  GraphicShininess=75  DoExposeReferenceFrame=on  SerializedFrames=<Frames/>
  Mark1 : sm_lib/Body Elements/Revolved Solid  RevolutionCrossSection=mark_xsec  RevolutionCrossSectionUnits=m  RevolutionExtent=Custom  RevolutionAngle=mark_angle_range  RevolutionAngleUnits=deg  ExportConvexHullGeometry=off  InertiaType=CalculateFromGeometry  BasedOnType=Density  Density=0  DensityUnits=kg/m^3  Mass=1  MassUnits=kg  CenterOfMass=[0 0 0]  CenterOfMassUnits=m  MomentsOfInertia=[1 1 1]  MomentsOfInertiaUnits=kg*m^2  ProductsOfInertia=[1 1 1]  ProductsOfInertiaUnits=kg*m^2  GraphicType=FromGeometry  MarkerShape=Sphere  MarkerSize=10  GraphicVisPropType=SimpleVisualProperties  GraphicDiffuseColor=mark_color  GraphicOpacity=mark_1_opc  GraphicSpecularColor=[0.5 0.5 0.5 1.0]  GraphicAmbientColor=[0.15 0.15 0.15 1.0]  GraphicEmissiveColor=[0.0 0.0 0.0 1.0]  GraphicShininess=75  DoExposeReferenceFrame=on  SerializedFrames=<Frames/>
  Mark2 : sm_lib/Body Elements/Revolved Solid  RevolutionCrossSection=mark_xsec  RevolutionCrossSectionUnits=m  RevolutionExtent=Custom  RevolutionAngle=mark_angle_range  RevolutionAngleUnits=deg  ExportConvexHullGeometry=off  InertiaType=CalculateFromGeometry  BasedOnType=Density  Density=0  DensityUnits=kg/m^3  Mass=1  MassUnits=kg  CenterOfMass=[0 0 0]  CenterOfMassUnits=m  MomentsOfInertia=[1 1 1]  MomentsOfInertiaUnits=kg*m^2  ProductsOfInertia=[1 1 1]  ProductsOfInertiaUnits=kg*m^2  GraphicType=FromGeometry  MarkerShape=Sphere  MarkerSize=10  GraphicVisPropType=SimpleVisualProperties  GraphicDiffuseColor=mark_color  GraphicOpacity=mark_2_opc  GraphicSpecularColor=[0.5 0.5 0.5 1.0]  GraphicAmbientColor=[0.15 0.15 0.15 1.0]  GraphicEmissiveColor=[0.0 0.0 0.0 1.0]  GraphicShininess=75  DoExposeReferenceFrame=on  SerializedFrames=<Frames/>
  Transform Mark2 : sm_lib/Frames and Transforms/Rigid Transform  RotationMethod=StandardAxis  FollAlignAxisA=+X  BaseAlignAxisA=+Y  FollAlignAxisB=+Y  BaseAlignAxisB=+Z  RotationStandardAxis=+Y  RotationAngle=180  RotationAngleUnits=deg  RotationArbitraryAxis=[0 0 1]  RotationSequenceAxes=FollowerAxes  RotationSequence=XYX  RotationSequenceAngles=[0 0 0]  RotationSequenceAnglesUnits=deg  RotationMatrix=[1 0 0; 0 1 0; 0 0 1]  Quaternion=[1 0 0 0]  TranslationMethod=None  TranslationCartesianOffset=[0 0 0]  TranslationCartesianOffsetUnits=m  TranslationStandardAxis=+Z  TranslationStandardOffset=0  TranslationStandardOffsetUnits=m  TranslationROffset=0  TranslationROffsetUnits=m  TranslationThetaOffset=0  TranslationThetaOffsetUnits=deg  TranslationZOffset=0  TranslationZOffsetUnits=m
  C : PMIOPort  Side=Right
  connections:
  Mark2/RConn1 -- Transform Mark2/RConn1
  Mark1/RConn1 -- Gear/RConn1 -- Transform Mark2/LConn1 -- C/RConn1

== system Multibody_Parts_Lib/Gears/Rack ==
  Rack : sm_lib/Body Elements/Extruded Solid  ExtrusionType=General  PolygonNumSides=3  PolygonOuterRadius=1  PolygonOuterRadiusUnits=m  ExportEntireGeometry=off  ExtrusionCrossSection=rack_xsec  ExtrusionCrossSectionUnits=m  ExportConvexHullGeometry=off  ExtrusionLength=rack_th  ExtrusionLengthUnits=m  InertiaType=CalculateFromGeometry  BasedOnType=Density  Density=rack_rho  DensityUnits=kg/(m^3)  Mass=1  MassUnits=kg  CenterOfMass=[0 0 0]  CenterOfMassUnits=m  MomentsOfInertia=[1 1 1]  MomentsOfInertiaUnits=kg*m^2  ProductsOfInertia=[0 0 0]  ProductsOfInertiaUnits=kg*m^2  GraphicType=FromGeometry  MarkerShape=Sphere  MarkerSize=10  GraphicVisPropType=SimpleVisualProperties  GraphicDiffuseColor=rack_clr  GraphicOpacity=rack_opc  GraphicSpecularColor=[0.5 0.5 0.5 1.0]  GraphicAmbientColor=[0.15 0.15 0.15 1.0]  GraphicEmissiveColor=[0.0 0.0 0.0 1.0]  GraphicShininess=75  DoExposeReferenceFrame=on  SerializedFrames=<Frames/>
  Transform Rack : sm_lib/Frames and Transforms/Rigid Transform  RotationMethod=StandardAxis  FollAlignAxisA=+X  BaseAlignAxisA=+Y  FollAlignAxisB=+Y  BaseAlignAxisB=+Z  RotationStandardAxis=+Y  RotationAngle=90  RotationAngleUnits=deg  RotationArbitraryAxis=[0 0 1]  RotationSequenceAxes=FollowerAxes  RotationSequence=XYX  RotationSequenceAngles=[0 0 0]  RotationSequenceAnglesUnits=deg  RotationMatrix=[1 0 0; 0 1 0; 0 0 1]  Quaternion=[1 0 0 0]  TranslationMethod=None  TranslationCartesianOffset=[0 0 0]  TranslationCartesianOffsetUnits=m  TranslationStandardAxis=+Z  TranslationStandardOffset=0  TranslationStandardOffsetUnits=m  TranslationROffset=0  TranslationROffsetUnits=m  TranslationThetaOffset=0  TranslationThetaOffsetUnits=deg  TranslationZOffset=0  TranslationZOffsetUnits=m
  C : PMIOPort  Side=Right
  connections:
  Transform Rack/LConn1 -- C/RConn1
  Transform Rack/RConn1 -- Rack/RConn1

== system Multibody_Parts_Lib/Linkages/Cam Circles ==
  Solid : sm_lib/Body Elements/Extruded Solid  ExtrusionType=General  PolygonNumSides=3  PolygonOuterRadius=1  PolygonOuterRadiusUnits=m  ExportEntireGeometry=off  ExtrusionCrossSection=cam_xsec  ExtrusionCrossSectionUnits=m  ExportConvexHullGeometry=off  ExtrusionLength=cam_thickness  ExtrusionLengthUnits=m  InertiaType=CalculateFromGeometry  BasedOnType=Density  Density=cam_rho  DensityUnits=kg/(m^3)  Mass=1  MassUnits=kg  CenterOfMass=[0 0 0]  CenterOfMassUnits=m  MomentsOfInertia=[1 1 1]  MomentsOfInertiaUnits=kg*m^2  ProductsOfInertia=[0 0 0]  ProductsOfInertiaUnits=kg*m^2  GraphicType=FromGeometry  MarkerShape=Sphere  MarkerSize=10  GraphicVisPropType=SimpleVisualProperties  GraphicDiffuseColor=cam_color  GraphicOpacity=cam_opc  GraphicSpecularColor=[0.5 0.5 0.5 1.0]  GraphicAmbientColor=[0.15 0.15 0.15 1.0]  GraphicEmissiveColor=[0.0 0.0 0.0 1.0]  GraphicShininess=75  DoExposeReferenceFrame=on  SerializedFrames=<Frames/>
  Transform pX : sm_lib/Frames and Transforms/Rigid Transform  RotationMethod=None  FollAlignAxisA=+X  BaseAlignAxisA=+Y  FollAlignAxisB=+Y  BaseAlignAxisB=+Z  RotationStandardAxis=+Z  RotationAngle=0.0  RotationAngleUnits=deg  RotationArbitraryAxis=[0 0 1]  RotationSequenceAxes=FollowerAxes  RotationSequence=XYX  RotationSequenceAngles=[0 0 0]  RotationSequenceAnglesUnits=deg  RotationMatrix=[1 0 0; 0 1 0; 0 0 1]  Quaternion=[1 0 0 0]  TranslationMethod=StandardAxis  TranslationCartesianOffset=[0 0 0]  TranslationCartesianOffsetUnits=m  TranslationStandardAxis=+X  TranslationStandardOffset=cam_len  TranslationStandardOffsetUnits=m  TranslationROffset=0  TranslationROffsetUnits=m  TranslationThetaOffset=0  TranslationThetaOffsetUnits=deg  TranslationZOffset=0  TranslationZOffsetUnits=m
  B : PMIOPort  Side=Left
  F : PMIOPort  Port=2  Side=Right
  connections:
  Transform pX/LConn1 -- Solid/RConn1 -- B/RConn1
  F/RConn1 -- Transform pX/RConn1

== system Multibody_Parts_Lib/Linkages/Link ==
  Solid : sm_lib/Body Elements/Extruded Solid  ExtrusionType=General  PolygonNumSides=3  PolygonOuterRadius=1  PolygonOuterRadiusUnits=m  ExportEntireGeometry=off  ExtrusionCrossSection=link_xsec  ExtrusionCrossSectionUnits=m  ExportConvexHullGeometry=off  ExtrusionLength=link_thickness  ExtrusionLengthUnits=m  InertiaType=CalculateFromGeometry  BasedOnType=Density  Density=link_rho  DensityUnits=kg/(m^3)  Mass=1  MassUnits=kg  CenterOfMass=[0 0 0]  CenterOfMassUnits=m  MomentsOfInertia=[1 1 1]  MomentsOfInertiaUnits=kg*m^2  ProductsOfInertia=[0 0 0]  ProductsOfInertiaUnits=kg*m^2  GraphicType=FromGeometry  MarkerShape=Sphere  MarkerSize=10  GraphicVisPropType=SimpleVisualProperties  GraphicDiffuseColor=link_color  GraphicOpacity=link_opc  GraphicSpecularColor=[0.5 0.5 0.5 1.0]  GraphicAmbientColor=[0.15 0.15 0.15 1.0]  GraphicEmissiveColor=[0.0 0.0 0.0 1.0]  GraphicShininess=75  DoExposeReferenceFrame=on  SerializedFrames=<Frames/>
  Transform B : sm_lib/Frames and Transforms/Rigid Transform  RotationMethod=None  FollAlignAxisA=+X  BaseAlignAxisA=+Y  FollAlignAxisB=+Y  BaseAlignAxisB=+Z  RotationStandardAxis=+Z  RotationAngle=0.0  RotationAngleUnits=deg  RotationArbitraryAxis=[0 0 1]  RotationSequenceAxes=FollowerAxes  RotationSequence=XYX  RotationSequenceAngles=[0 0 0]  RotationSequenceAnglesUnits=deg  RotationMatrix=[1 0 0; 0 1 0; 0 0 1]  Quaternion=[1 0 0 0]  TranslationMethod=StandardAxis  TranslationCartesianOffset=[0 0 0]  TranslationCartesianOffsetUnits=m  TranslationStandardAxis=-X  TranslationStandardOffset=link_len/2  TranslationStandardOffsetUnits=m  TranslationROffset=0  TranslationROffsetUnits=m  TranslationThetaOffset=0  TranslationThetaOffsetUnits=deg  TranslationZOffset=0  TranslationZOffsetUnits=m
  Transform F : sm_lib/Frames and Transforms/Rigid Transform  RotationMethod=None  FollAlignAxisA=+X  BaseAlignAxisA=+Y  FollAlignAxisB=+Y  BaseAlignAxisB=+Z  RotationStandardAxis=+Z  RotationAngle=0.0  RotationAngleUnits=deg  RotationArbitraryAxis=[0 0 1]  RotationSequenceAxes=FollowerAxes  RotationSequence=XYX  RotationSequenceAngles=[0 0 0]  RotationSequenceAnglesUnits=deg  RotationMatrix=[1 0 0; 0 1 0; 0 0 1]  Quaternion=[1 0 0 0]  TranslationMethod=StandardAxis  TranslationCartesianOffset=[0 0 0]  TranslationCartesianOffsetUnits=m  TranslationStandardAxis=+X  TranslationStandardOffset=link_len/2  TranslationStandardOffsetUnits=m  TranslationROffset=0  TranslationROffsetUnits=m  TranslationThetaOffset=0  TranslationThetaOffsetUnits=deg  TranslationZOffset=0  TranslationZOffsetUnits=m
  F : PMIOPort  Side=Right
  B : PMIOPort  Port=2  Side=Left
  connections:
  Solid/RConn1 -- Transform F/LConn1 -- Transform B/LConn1
  Transform B/RConn1 -- B/RConn1
  Transform F/RConn1 -- F/RConn1

== system Multibody_Parts_Lib/Linkages/Link End ==
  Solid : sm_lib/Body Elements/Extruded Solid  ExtrusionType=General  PolygonNumSides=3  PolygonOuterRadius=1  PolygonOuterRadiusUnits=m  ExportEntireGeometry=off  ExtrusionCrossSection=circ_xsec  ExtrusionCrossSectionUnits=m  ExportConvexHullGeometry=off  ExtrusionLength=circ_len  ExtrusionLengthUnits=m  InertiaType=CalculateFromGeometry  BasedOnType=Density  Density=circ_rho  DensityUnits=kg/(m^3)  Mass=1  MassUnits=kg  CenterOfMass=[0 0 0]  CenterOfMassUnits=m  MomentsOfInertia=[1 1 1]  MomentsOfInertiaUnits=kg*m^2  ProductsOfInertia=[0 0 0]  ProductsOfInertiaUnits=kg*m^2  GraphicType=FromGeometry  MarkerShape=Sphere  MarkerSize=10  GraphicVisPropType=SimpleVisualProperties  GraphicDiffuseColor=circ_color  GraphicOpacity=circ_opc  GraphicSpecularColor=[0.5 0.5 0.5 1.0]  GraphicAmbientColor=[0.15 0.15 0.15 1.0]  GraphicEmissiveColor=[0.0 0.0 0.0 1.0]  GraphicShininess=75  DoExposeReferenceFrame=on  SerializedFrames=<Frames/>
  Transform B : sm_lib/Frames and Transforms/Rigid Transform  RotationMethod=StandardAxis  FollAlignAxisA=+X  BaseAlignAxisA=+Y  FollAlignAxisB=+Y  BaseAlignAxisB=+Z  RotationStandardAxis=+Y  RotationAngle=0  RotationAngleUnits=deg  RotationArbitraryAxis=[0 0 1]  RotationSequenceAxes=FollowerAxes  RotationSequence=XYX  RotationSequenceAngles=[0 0 0]  RotationSequenceAnglesUnits=deg  RotationMatrix=[1 0 0; 0 1 0; 0 0 1]  Quaternion=[1 0 0 0]  TranslationMethod=None  TranslationCartesianOffset=[0 0 0]  TranslationCartesianOffsetUnits=m  TranslationStandardAxis=+X  TranslationStandardOffset=0  TranslationStandardOffsetUnits=m  TranslationROffset=0  TranslationROffsetUnits=m  TranslationThetaOffset=0  TranslationThetaOffsetUnits=deg  TranslationZOffset=0  TranslationZOffsetUnits=m
  X : PMIOPort  Side=Left
  connections:
  Transform B/RConn1 -- Solid/RConn1
  Transform B/LConn1 -- X/RConn1
